simulink model "Simscape_Drone_Model"  (R2025b)
settings: Solver=FixedStepAuto  StartTime=0.0  StopTime=10  RelTol=1e-6  EnableMultiTasking=on
undefined symbols (not defined in the file): Aero_On, Config, P, SimParams, SimscapeParams, X, Y, Z
libraries: sm_lib x89, nesl_utility x71, fl_lib x18, sdl_lib x8, slpidlib x4, batteryecm_lib x1
(part 5 of 5)

== system Simscape_Drone_Model/Drone Mechanical/Motor Holder 4/Aero Dynamic Drag ==
  rho : Inport
  Gain : Gain  Gain=Aero_On
  MATLAB Function : MATLAB Function  TreatAsAtomicUnit=on
  Motor Holder Axis : Constant  Value=SimscapeParams.MotorHolderAxis
  Motor Holder Drag Matrix : Constant  Value=SimscapeParams.MotorHolderCd
  Motor Holder Length : Constant  Value=SimscapeParams.MotorHeight
  Motor Holder Radius : Constant  Value=SimscapeParams.MotorRadius
  Mux : Mux  Inputs=3
  PS-Simulink Converter : nesl_utility/PS-Simulink Converter  PhysicalDomain=network_engine_domain  SubClassName=ps_output  LeftPortType=input  RightPortType=output  PseudoPeriodic=off  Frequencies=[]  VectorFormat=inherit  Unit=inherit  AffineConversion=off
  PS-Simulink Converter1 : nesl_utility/PS-Simulink Converter  PhysicalDomain=network_engine_domain  SubClassName=ps_output  LeftPortType=input  RightPortType=output  PseudoPeriodic=off  Frequencies=[]  VectorFormat=inherit  Unit=inherit  AffineConversion=off
  PS-Simulink Converter2 : nesl_utility/PS-Simulink Converter  PhysicalDomain=network_engine_domain  SubClassName=ps_output  LeftPortType=input  RightPortType=output  PseudoPeriodic=off  Frequencies=[]  VectorFormat=inherit  Unit=inherit  AffineConversion=off
  Transform Sensor : sm_lib/Frames and Transforms/Transform Sensor  MeasurementFrame=NonRotatingFollower  RotationSequence=XYZ  SenseAngle=off  SenseAxis=off  SenseQ=off  SenseR=off  SenseRotationSequence=off  SenseOmegaX=off  SenseOmegaY=off  SenseOmegaZ=off  SenseOmega=off  SenseQDot=off  SenseRDot=off  SenseRotationSequenceDot=off  SenseAlphaX=off  SenseAlphaY=off  SenseAlphaZ=off  SenseAlpha=off  SenseQDDot=off  SenseRDDot=off  SenseX=off  SenseY=off  SenseZ=off  SenseXYZ=off  SenseRad=off  SenseAzim=off  SenseDist=off  SenseInc=off  SenseXDot=on  SenseYDot=on  SenseZDot=on  SenseXYZDot=off  SenseRadDot=off  SenseAzimDot=off  SenseDistDot=off  SenseIncDot=off  SenseXDDot=off  SenseYDDot=off  SenseZDDot=off  SenseXYZDDot=off  SenseRadDDot=off  SenseAzimDDot=off  SenseDistDDot=off  SenseIncDDot=off
  NED : PMIOPort  Side=Left
  F : PMIOPort  Port=2  Side=Left
  F_drag : Outport
  wires:
  PS-Simulink Converter/1 -> Mux/1
  PS-Simulink Converter2/1 -> Mux/3
  PS-Simulink Converter1/1 -> Mux/2
  rho/1 -> MATLAB Function/2(rho)
  Motor Holder Drag Matrix/1 -> MATLAB Function/3(Cd)
  Motor Holder Axis/1 -> MATLAB Function/6(axis)
  Motor Holder Radius/1 -> MATLAB Function/4(R)
  Motor Holder Length/1 -> MATLAB Function/5(L)
  Mux/1 -> MATLAB Function/1(v)
  MATLAB Function/1(F_drag) -> Gain/1
  Gain/1 -> F_drag/1
  connections:
  PS-Simulink Converter1/LConn1 -- Transform Sensor/RConn3
  PS-Simulink Converter2/LConn1 -- Transform Sensor/RConn4
  PS-Simulink Converter/LConn1 -- Transform Sensor/RConn2
  NED/RConn1 -- Transform Sensor/LConn1
  F/RConn1 -- Transform Sensor/RConn1

== system Simscape_Drone_Model/Drone Mechanical/Rotor arms/Subsystem ==
  note: Aero Dynamic Drag 2
  rho : Inport
  Arm Axis : Constant  Value=SimscapeParams.ArmAxis
  Arm Drag Matrix : Constant  Value=SimscapeParams.ArmCd
  Arm Length : Constant  Value=SimscapeParams.ArmLength
  Arm Radius : Constant  Value=SimscapeParams.ArmRadius
  Gain : Gain  Gain=Aero_On
  MATLAB Function : MATLAB Function  TreatAsAtomicUnit=on
  Mux : Mux  Inputs=3
  PS-Simulink Converter : nesl_utility/PS-Simulink Converter  PhysicalDomain=network_engine_domain  SubClassName=ps_output  LeftPortType=input  RightPortType=output  PseudoPeriodic=off  Frequencies=[]  VectorFormat=inherit  Unit=inherit  AffineConversion=off
  PS-Simulink Converter1 : nesl_utility/PS-Simulink Converter  PhysicalDomain=network_engine_domain  SubClassName=ps_output  LeftPortType=input  RightPortType=output  PseudoPeriodic=off  Frequencies=[]  VectorFormat=inherit  Unit=inherit  AffineConversion=off
  PS-Simulink Converter2 : nesl_utility/PS-Simulink Converter  PhysicalDomain=network_engine_domain  SubClassName=ps_output  LeftPortType=input  RightPortType=output  PseudoPeriodic=off  Frequencies=[]  VectorFormat=inherit  Unit=inherit  AffineConversion=off
  Transform Sensor : sm_lib/Frames and Transforms/Transform Sensor  MeasurementFrame=NonRotatingFollower  RotationSequence=XYZ  SenseAngle=off  SenseAxis=off  SenseQ=off  SenseR=off  SenseRotationSequence=off  SenseOmegaX=off  SenseOmegaY=off  SenseOmegaZ=off  SenseOmega=off  SenseQDot=off  SenseRDot=off  SenseRotationSequenceDot=off  SenseAlphaX=off  SenseAlphaY=off  SenseAlphaZ=off  SenseAlpha=off  SenseQDDot=off  SenseRDDot=off  SenseX=off  SenseY=off  SenseZ=off  SenseXYZ=off  SenseRad=off  SenseAzim=off  SenseDist=off  SenseInc=off  SenseXDot=on  SenseYDot=on  SenseZDot=on  SenseXYZDot=off  SenseRadDot=off  SenseAzimDot=off  SenseDistDot=off  SenseIncDot=off  SenseXDDot=off  SenseYDDot=off  SenseZDDot=off  SenseXYZDDot=off  SenseRadDDot=off  SenseAzimDDot=off  SenseDistDDot=off  SenseIncDDot=off
  NED : PMIOPort  Side=Left
  F : PMIOPort  Port=2  Side=Right
  F_drag : Outport
  wires:
  MATLAB Function/1(F_drag) -> Gain/1
  Mux/1 -> MATLAB Function/1(v)
  PS-Simulink Converter/1 -> Mux/1
  Arm Length/1 -> MATLAB Function/5(L)
  rho/1 -> MATLAB Function/2(rho)
  Arm Drag Matrix/1 -> MATLAB Function/3(Cd)
  PS-Simulink Converter2/1 -> Mux/3
  Arm Radius/1 -> MATLAB Function/4(R)
  PS-Simulink Converter1/1 -> Mux/2
  Arm Axis/1 -> MATLAB Function/6(axis)
  Gain/1 -> F_drag/1
  connections:
  PS-Simulink Converter/LConn1 -- Transform Sensor/RConn2
  PS-Simulink Converter1/LConn1 -- Transform Sensor/RConn3
  NED/RConn1 -- Transform Sensor/LConn1
  PS-Simulink Converter2/LConn1 -- Transform Sensor/RConn4
  F/RConn1 -- Transform Sensor/RConn1

== system Simscape_Drone_Model/Drone Mechanical/Rotor arms/Subsystem1 ==
  note: Aero Dynamic Drag 1
  rho : Inport
  Arm Axis : Constant  Value=SimscapeParams.ArmAxis
  Arm Drag Matrix : Constant  Value=SimscapeParams.ArmCd
  Arm Length : Constant  Value=SimscapeParams.ArmLength
  Arm Radius : Constant  Value=SimscapeParams.ArmRadius
  Gain : Gain  Gain=Aero_On
  MATLAB Function : MATLAB Function  TreatAsAtomicUnit=on
  Mux : Mux  Inputs=3
  PS-Simulink Converter : nesl_utility/PS-Simulink Converter  PhysicalDomain=network_engine_domain  SubClassName=ps_output  LeftPortType=input  RightPortType=output  PseudoPeriodic=off  Frequencies=[]  VectorFormat=inherit  Unit=inherit  AffineConversion=off
  PS-Simulink Converter1 : nesl_utility/PS-Simulink Converter  PhysicalDomain=network_engine_domain  SubClassName=ps_output  LeftPortType=input  RightPortType=output  PseudoPeriodic=off  Frequencies=[]  VectorFormat=inherit  Unit=inherit  AffineConversion=off
  PS-Simulink Converter2 : nesl_utility/PS-Simulink Converter  PhysicalDomain=network_engine_domain  SubClassName=ps_output  LeftPortType=input  RightPortType=output  PseudoPeriodic=off  Frequencies=[]  VectorFormat=inherit  Unit=inherit  AffineConversion=off
  Transform Sensor : sm_lib/Frames and Transforms/Transform Sensor  MeasurementFrame=NonRotatingFollower  RotationSequence=XYZ  SenseAngle=off  SenseAxis=off  SenseQ=off  SenseR=off  SenseRotationSequence=off  SenseOmegaX=off  SenseOmegaY=off  SenseOmegaZ=off  SenseOmega=off  SenseQDot=off  SenseRDot=off  SenseRotationSequenceDot=off  SenseAlphaX=off  SenseAlphaY=off  SenseAlphaZ=off  SenseAlpha=off  SenseQDDot=off  SenseRDDot=off  SenseX=off  SenseY=off  SenseZ=off  SenseXYZ=off  SenseRad=off  SenseAzim=off  SenseDist=off  SenseInc=off  SenseXDot=on  SenseYDot=on  SenseZDot=on  SenseXYZDot=off  SenseRadDot=off  SenseAzimDot=off  SenseDistDot=off  SenseIncDot=off  SenseXDDot=off  SenseYDDot=off  SenseZDDot=off  SenseXYZDDot=off  SenseRadDDot=off  SenseAzimDDot=off  SenseDistDDot=off  SenseIncDDot=off
  NED : PMIOPort  Side=Left
  F : PMIOPort  Port=2  Side=Right
  F_drag : Outport
  wires:
  MATLAB Function/1(F_drag) -> Gain/1
  Mux/1 -> MATLAB Function/1(v)
  PS-Simulink Converter/1 -> Mux/1
  Arm Length/1 -> MATLAB Function/5(L)
  rho/1 -> MATLAB Function/2(rho)
  Arm Drag Matrix/1 -> MATLAB Function/3(Cd)
  PS-Simulink Converter2/1 -> Mux/3
  Arm Radius/1 -> MATLAB Function/4(R)
  PS-Simulink Converter1/1 -> Mux/2
  Arm Axis/1 -> MATLAB Function/6(axis)
  Gain/1 -> F_drag/1
  connections:
  PS-Simulink Converter/LConn1 -- Transform Sensor/RConn2
  PS-Simulink Converter1/LConn1 -- Transform Sensor/RConn3
  NED/RConn1 -- Transform Sensor/LConn1
  PS-Simulink Converter2/LConn1 -- Transform Sensor/RConn4
  F/RConn1 -- Transform Sensor/RConn1

== system Simscape_Drone_Model/Drone Mechanical/Rotor arms/Subsystem2 ==
  note: Aero Dynamic Drag 4
  rho : Inport
  Arm Axis : Constant  Value=SimscapeParams.ArmAxis
  Arm Drag Matrix : Constant  Value=SimscapeParams.ArmCd
  Arm Length : Constant  Value=SimscapeParams.ArmLength
  Arm Radius : Constant  Value=SimscapeParams.ArmRadius
  Gain : Gain  Gain=Aero_On
  MATLAB Function : MATLAB Function  TreatAsAtomicUnit=on
  Mux : Mux  Inputs=3
  PS-Simulink Converter : nesl_utility/PS-Simulink Converter  PhysicalDomain=network_engine_domain  SubClassName=ps_output  LeftPortType=input  RightPortType=output  PseudoPeriodic=off  Frequencies=[]  VectorFormat=inherit  Unit=inherit  AffineConversion=off
  PS-Simulink Converter1 : nesl_utility/PS-Simulink Converter  PhysicalDomain=network_engine_domain  SubClassName=ps_output  LeftPortType=input  RightPortType=output  PseudoPeriodic=off  Frequencies=[]  VectorFormat=inherit  Unit=inherit  AffineConversion=off
  PS-Simulink Converter2 : nesl_utility/PS-Simulink Converter  PhysicalDomain=network_engine_domain  SubClassName=ps_output  LeftPortType=input  RightPortType=output  PseudoPeriodic=off  Frequencies=[]  VectorFormat=inherit  Unit=inherit  AffineConversion=off
  Transform Sensor : sm_lib/Frames and Transforms/Transform Sensor  MeasurementFrame=NonRotatingFollower  RotationSequence=XYZ  SenseAngle=off  SenseAxis=off  SenseQ=off  SenseR=off  SenseRotationSequence=off  SenseOmegaX=off  SenseOmegaY=off  SenseOmegaZ=off  SenseOmega=off  SenseQDot=off  SenseRDot=off  SenseRotationSequenceDot=off  SenseAlphaX=off  SenseAlphaY=off  SenseAlphaZ=off  SenseAlpha=off  SenseQDDot=off  SenseRDDot=off  SenseX=off  SenseY=off  SenseZ=off  SenseXYZ=off  SenseRad=off  SenseAzim=off  SenseDist=off  SenseInc=off  SenseXDot=on  SenseYDot=on  SenseZDot=on  SenseXYZDot=off  SenseRadDot=off  SenseAzimDot=off  SenseDistDot=off  SenseIncDot=off  SenseXDDot=off  SenseYDDot=off  SenseZDDot=off  SenseXYZDDot=off  SenseRadDDot=off  SenseAzimDDot=off  SenseDistDDot=off  SenseIncDDot=off
  NED : PMIOPort  Side=Left
  F : PMIOPort  Port=2  Side=Right
  F_drag : Outport
  wires:
  MATLAB Function/1(F_drag) -> Gain/1
  Mux/1 -> MATLAB Function/1(v)
  PS-Simulink Converter/1 -> Mux/1
  Arm Length/1 -> MATLAB Function/5(L)
  rho/1 -> MATLAB Function/2(rho)
  Arm Drag Matrix/1 -> MATLAB Function/3(Cd)
  PS-Simulink Converter2/1 -> Mux/3
  Arm Radius/1 -> MATLAB Function/4(R)
  PS-Simulink Converter1/1 -> Mux/2
  Arm Axis/1 -> MATLAB Function/6(axis)
  Gain/1 -> F_drag/1
  connections:
  PS-Simulink Converter/LConn1 -- Transform Sensor/RConn2
  PS-Simulink Converter1/LConn1 -- Transform Sensor/RConn3
  NED/RConn1 -- Transform Sensor/LConn1
  PS-Simulink Converter2/LConn1 -- Transform Sensor/RConn4
  F/RConn1 -- Transform Sensor/RConn1

== system Simscape_Drone_Model/Drone Mechanical/Rotor arms/Subsystem3 ==
  note: Aero Dynamic Drag 3
  rho : Inport
  Arm Axis : Constant  Value=SimscapeParams.ArmAxis
  Arm Drag Matrix : Constant  Value=SimscapeParams.ArmCd
  Arm Length : Constant  Value=SimscapeParams.ArmLength
  Arm Radius : Constant  Value=SimscapeParams.ArmRadius
  Gain : Gain  Gain=Aero_On
  MATLAB Function : MATLAB Function  TreatAsAtomicUnit=on
  Mux : Mux  Inputs=3
  PS-Simulink Converter : nesl_utility/PS-Simulink Converter  PhysicalDomain=network_engine_domain  SubClassName=ps_output  LeftPortType=input  RightPortType=output  PseudoPeriodic=off  Frequencies=[]  VectorFormat=inherit  Unit=inherit  AffineConversion=off
  PS-Simulink Converter1 : nesl_utility/PS-Simulink Converter  PhysicalDomain=network_engine_domain  SubClassName=ps_output  LeftPortType=input  RightPortType=output  PseudoPeriodic=off  Frequencies=[]  VectorFormat=inherit  Unit=inherit  AffineConversion=off
  PS-Simulink Converter2 : nesl_utility/PS-Simulink Converter  PhysicalDomain=network_engine_domain  SubClassName=ps_output  LeftPortType=input  RightPortType=output  PseudoPeriodic=off  Frequencies=[]  VectorFormat=inherit  Unit=inherit  AffineConversion=off
  Transform Sensor : sm_lib/Frames and Transforms/Transform Sensor  MeasurementFrame=NonRotatingFollower  RotationSequence=XYZ  SenseAngle=off  SenseAxis=off  SenseQ=off  SenseR=off  SenseRotationSequence=off  SenseOmegaX=off  SenseOmegaY=off  SenseOmegaZ=off  SenseOmega=off  SenseQDot=off  SenseRDot=off  SenseRotationSequenceDot=off  SenseAlphaX=off  SenseAlphaY=off  SenseAlphaZ=off  SenseAlpha=off  SenseQDDot=off  SenseRDDot=off  SenseX=off  SenseY=off  SenseZ=off  SenseXYZ=off  SenseRad=off  SenseAzim=off  SenseDist=off  SenseInc=off  SenseXDot=on  SenseYDot=on  SenseZDot=on  SenseXYZDot=off  SenseRadDot=off  SenseAzimDot=off  SenseDistDot=off  SenseIncDot=off  SenseXDDot=off  SenseYDDot=off  SenseZDDot=off  SenseXYZDDot=off  SenseRadDDot=off  SenseAzimDDot=off  SenseDistDDot=off  SenseIncDDot=off
  NED : PMIOPort  Side=Left
  F : PMIOPort  Port=2  Side=Right
  F_drag : Outport
  wires:
  MATLAB Function/1(F_drag) -> Gain/1
  Mux/1 -> MATLAB Function/1(v)
  PS-Simulink Converter/1 -> Mux/1
  Arm Length/1 -> MATLAB Function/5(L)
  rho/1 -> MATLAB Function/2(rho)
  Arm Drag Matrix/1 -> MATLAB Function/3(Cd)
  PS-Simulink Converter2/1 -> Mux/3
  Arm Radius/1 -> MATLAB Function/4(R)
  PS-Simulink Converter1/1 -> Mux/2
  Arm Axis/1 -> MATLAB Function/6(axis)
  Gain/1 -> F_drag/1
  connections:
  PS-Simulink Converter/LConn1 -- Transform Sensor/RConn2
  PS-Simulink Converter1/LConn1 -- Transform Sensor/RConn3
  NED/RConn1 -- Transform Sensor/LConn1
  PS-Simulink Converter2/LConn1 -- Transform Sensor/RConn4
  F/RConn1 -- Transform Sensor/RConn1

== system Simscape_Drone_Model/Drone Mechanical/Body/Top Payload/Top Payload ==
  rho : Inport
  Collsioin : Subsystem
  Cylindrical Solid : sm_lib/Body Elements/Cylindrical Solid  CylinderRadius=Config.TopPayload.Geometry.Radius  CylinderRadiusUnits=m  CylinderLength=Config.TopPayload.Geometry.Height  CylinderLengthUnits=m  ExportEntireGeometry=off  InertiaType=CalculateFromGeometry  BasedOnType=Mass  Density=1000  DensityUnits=kg/m^3  Mass=Config.TopPayload.Mass  MassUnits=kg  CenterOfMass=[0 0 0]  CenterOfMassUnits=m  MomentsOfInertia=[1 1 1]  MomentsOfInertiaUnits=kg*m^2  ProductsOfInertia=[0 0 0]  ProductsOfInertiaUnits=kg*m^2  GraphicType=FromGeometry  MarkerShape=Sphere  MarkerSize=10  GraphicVisPropType=SimpleVisualProperties  GraphicDiffuseColor=[1 0 1]  GraphicOpacity=1  GraphicSpecularColor=[0.5 0.5 0.5 1.0]  GraphicAmbientColor=[0.15 0.15 0.15 1.0]  GraphicEmissiveColor=[0.0 0.0 0.0 1.0]  GraphicShininess=75  DoExposeReferenceFrame=on  SerializedFrames=|
      | <Frames>
      | 
      |   <Frame>
      |     <Id>Frame1</Id>
      |     <Value>
      |       <Name>side</Name>
      |       <Origin>
      |         <Source>GeometricFeature</Source>
      |         <FeatureName>side surface</FeatureName>
      |       </Origin>
      |       <PrimaryAxis>
      |         <DefinedDirection>+Z</DefinedDirection>
      |         <Source>ReferenceFrame</Source>
      |         <SourceDirection>+Z</SourceDirection>
      |         <FeatureName></FeatureName>
      |       </PrimaryAxis>
      |       <SecondaryAxis>
      |         <DefinedDirection>+X</DefinedDirection>
      |         <Source>ReferenceFrame</Source>
      |         <SourceDirection>+X</SourceDirection>
      |         <FeatureName></FeatureName>
      |       </SecondaryAxis>
      |     </Value>
      |   </Frame>
      | 
      | </Frames>
  External Force and Torque1 : sm_lib/Forces and Torques/External Force and Torque  EnableForceX=off  EnableForceY=off  EnableForceZ=off  EnableForce=on  ForceResolutionFrame=AttachedFrame  EnableTorqueX=off  EnableTorqueY=off  EnableTorqueZ=off  EnableTorque=off  TorqueResolutionFrame=AttachedFrame
  Rigid Transform : sm_lib/Frames and Transforms/Rigid Transform  RotationMethod=None  FollAlignAxisA=+X  BaseAlignAxisA=+Y  FollAlignAxisB=+Y  BaseAlignAxisB=+Z  RotationStandardAxis=+Z  RotationAngle=0  RotationAngleUnits=deg  RotationArbitraryAxis=[0 0 1]  RotationSequenceAxes=FollowerAxes  RotationSequence=XYX  RotationSequenceAngles=[0 0 0]  RotationSequenceAnglesUnits=deg  RotationMatrix=[1 0 0;0 1 0;0 0 1]  Quaternion=[1 0 0 0]  TranslationMethod=Cartesian  TranslationCartesianOffset=[0 0 -(Config.Drone.Body_Height/2 + Config.TopPayload.Geometry.Height/2)]  TranslationCartesianOffsetUnits=m  TranslationStandardAxis=+Z  TranslationStandardOffset=0  TranslationStandardOffsetUnits=m  TranslationROffset=0  TranslationROffsetUnits=m  TranslationThetaOffset=0  TranslationThetaOffsetUnits=deg  TranslationZOffset=0  TranslationZOffsetUnits=m
  Simulink-PS Converter1 : nesl_utility/Simulink-PS Converter  PhysicalDomain=network_engine_domain  SubClassName=ps_input  LeftPortType=input  RightPortType=output  PseudoPeriodic=off  Frequencies=[]  NoiseDistribution=none  NoiseParameters=[]  Unit=N  AffineConversion=off  FilteringAndDerivatives=provide  SimscapeFilterOrder=1  InputFilterTimeConstant=0.001  UdotUserProvided=0
  Top payload drag : Subsystem
      settings: PortSchema="{\"entries\":[{\"content\":{\"sides\":[{\"content\":{\"connectorIds\":[\"LConn1\",\"In1\"]},\"type\":\"ConnectorPlacement.EquallySpacedRectSide\",\"uuid\":\"0fc06b31-134b-40cc-bbcb-bc6e67fd0f90\"},{\"content\":{\"connectorIds\":[\"RConn1\",\"Out1\"],\"side\":\"RIGHT\"},\"type\":\"ConnectorPlacement.EquallySpacedRectSide\",\"uuid\":\"8ba8f1df-0f30-4005-8c63-0e1ae2e2ce41\"},{\"content\":{\"side\":\"TOP\"},\"type\":\"ConnectorPlacement.EquallySpacedRectSide\",\"uuid\":\"8c63a784-8cbe-42b9-959e-29358ae8c9e6\"}]},\"type\":\"ConnectorPlacement.EquallySpacedConnector\",\"uuid\":\"fa01ef64-01b6-4a76-afbb-3e89d462b0f0\"}],\"packageUris\":[\"http://schema.mathworks.com/mf0/Connector/R2020b\"],\"version\":\"1.0\"}"
  Top Connection : PMIOPort  Side=Left
  NED : PMIOPort  Port=2  Side=Left
  Body Collision : PMIOPort  Port=3  Side=Left
  wires:
  Top payload drag/1(F_drag) -> Simulink-PS Converter1/1
  rho/1 -> Top payload drag/1(rho)
  connections:
  External Force and Torque1/LConn1 -- Simulink-PS Converter1/RConn1
  Cylindrical Solid/RConn1 -- Rigid Transform/RConn1 -- External Force and Torque1/RConn1 -- Top payload drag/RConn1
  Rigid Transform/LConn1 -- Top Connection/RConn1
  Top payload drag/LConn1 -- NED/RConn1
  Collsioin/LConn1 -- Cylindrical Solid/LConn1
  Body Collision/RConn1 -- Collsioin/RConn1

== system Simscape_Drone_Model/Drone Mechanical/Body/Top Payload/Top Payload/Collsioin ==
  PS-Simulink Converter : nesl_utility/PS-Simulink Converter  PhysicalDomain=network_engine_domain  SubClassName=ps_output  LeftPortType=input  RightPortType=output  PseudoPeriodic=off  Frequencies=[]  VectorFormat=inherit  Unit=inherit  AffineConversion=off
  PS-Simulink Converter1 : nesl_utility/PS-Simulink Converter  PhysicalDomain=network_engine_domain  SubClassName=ps_output  LeftPortType=input  RightPortType=output  PseudoPeriodic=off  Frequencies=[]  VectorFormat=inherit  Unit=inherit  AffineConversion=off
  PS-Simulink Converter2 : nesl_utility/PS-Simulink Converter  PhysicalDomain=network_engine_domain  SubClassName=ps_output  LeftPortType=input  RightPortType=output  PseudoPeriodic=off  Frequencies=[]  VectorFormat=inherit  Unit=inherit  AffineConversion=off
  Point Cloud : sm_lib/Curves and Surfaces/Point Cloud  CoordinatesMatrix=SimscapeParams.TopPayloadSurfacePoints  CoordinatesMatrixUnits=m  GraphicType=MarkerCloud  GraphicSphereRadius=1e-2  GraphicSphereRadiusUnits=m  GraphicVisPropType=SimpleVisualProperties  GraphicDiffuseColor=[0.5 0.5 0.5]  GraphicOpacity=1  GraphicSpecularColor=[0.5 0.5 0.5 1.0]  GraphicAmbientColor=[0.15 0.15 0.15 1.0]  GraphicEmissiveColor=[0.0 0.0 0.0 1.0]  GraphicShininess=75
  Scope : Scope  Commented=on  NumInputPorts=3
      settings: ActiveDisplayYMinimum=-0.12499999999999997  ActiveDisplayYMaximum=1.125  DataLoggingVariableName=ScopeData3
  Spatial Contact Force1 : sm_lib/Forces and Torques/Spatial Contact Force  SenseSeparationDistance=off  NormalForceType=SmoothSpringDamper  NormalStiffness=2.5e4  NormalStiffnessUnits=N/m  NormalDamping=50  NormalDampingUnits=N/(m/s)  NormalTransitionRegionWidth=1e-3  NormalTransitionRegionWidthUnits=m  FrictionType=None  CoefficientOfStaticFriction=0.8  CoefficientOfDynamicFriction=0.5  FrictionalCriticalVelocity=1e-2  FrictionalCriticalVelocityUnits=m/s  SenseContactSignal=on  SensePenetrationDepth=off  SenseNormalVelocity=off  SenseTangentialVelocity=on  SensingForceTorqueDirection=BaseOnFollower  SensingForceTorqueResolutionFrame=BaseFrame  SenseNormalForce=off  SenseNormalForceMagnitude=off  SenseNormalTorque=off  SenseFrictionalForce=on  SenseFrictionalForceMagnitude=off  SenseFrictionalTorque=off  SenseTotalForce=off  SenseTotalTorque=off  SenseContactBaseRotation=off  SenseContactBaseTranslation=off  SenseContactFollowerRotation=off  SenseContactFollowerTranslation=off  ZeroCrossDetectContactStartAndEnd=off
  Side : PMIOPort  Side=Left
  Body Collision : PMIOPort  Port=2  Side=Right
  wires:
  PS-Simulink Converter2/1 -> Scope/3  "Tangential Velocity"
  PS-Simulink Converter1/1 -> Scope/2  "Frictional Force"
  PS-Simulink Converter/1 -> Scope/1  "Contact"
  connections:
  PS-Simulink Converter2/LConn1 -- Spatial Contact Force1/RConn4
  PS-Simulink Converter1/LConn1 -- Spatial Contact Force1/RConn3
  PS-Simulink Converter/LConn1 -- Spatial Contact Force1/RConn2
  Side/RConn1 -- Point Cloud/LConn1
  Spatial Contact Force1/LConn1 -- Point Cloud/RConn1
  Spatial Contact Force1/RConn1 -- Body Collision/RConn1

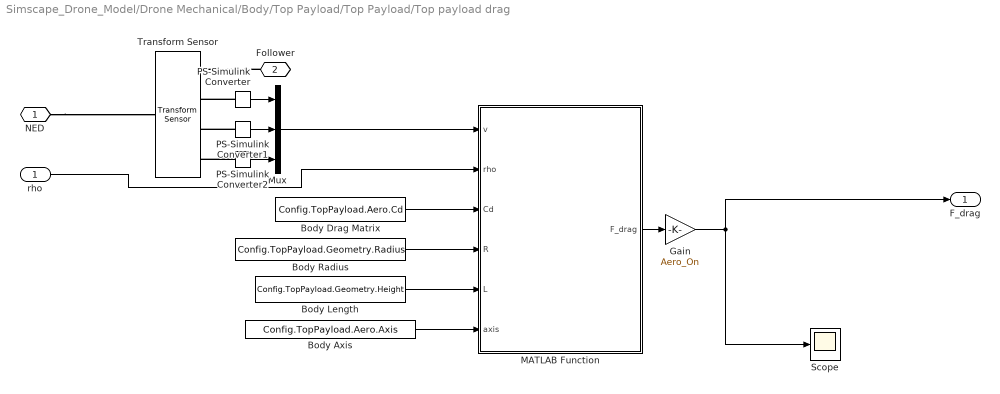
== system Simscape_Drone_Model/Drone Mechanical/Body/Top Payload/Top Payload/Top payload drag ==
  rho : Inport
  Body Axis : Constant  Value=Config.TopPayload.Aero.Axis
  Body Drag Matrix : Constant  Value=Config.TopPayload.Aero.Cd
  Body Length : Constant  Value=Config.TopPayload.Geometry.Height
  Body Radius : Constant  Value=Config.TopPayload.Geometry.Radius
  Gain : Gain  Gain=Aero_On
  MATLAB Function : MATLAB Function  TreatAsAtomicUnit=on
  Mux : Mux  Inputs=3
  PS-Simulink Converter : nesl_utility/PS-Simulink Converter  PhysicalDomain=network_engine_domain  SubClassName=ps_output  LeftPortType=input  RightPortType=output  PseudoPeriodic=off  Frequencies=[]  VectorFormat=inherit  Unit=inherit  AffineConversion=off
  PS-Simulink Converter1 : nesl_utility/PS-Simulink Converter  PhysicalDomain=network_engine_domain  SubClassName=ps_output  LeftPortType=input  RightPortType=output  PseudoPeriodic=off  Frequencies=[]  VectorFormat=inherit  Unit=inherit  AffineConversion=off
  PS-Simulink Converter2 : nesl_utility/PS-Simulink Converter  PhysicalDomain=network_engine_domain  SubClassName=ps_output  LeftPortType=input  RightPortType=output  PseudoPeriodic=off  Frequencies=[]  VectorFormat=inherit  Unit=inherit  AffineConversion=off
  Scope : Scope
      settings: ActiveDisplayYMinimum=-1  ActiveDisplayYMaximum=1  DataLoggingVariableName=ScopeData4
  Transform Sensor : sm_lib/Frames and Transforms/Transform Sensor  MeasurementFrame=NonRotatingFollower  RotationSequence=XYZ  SenseAngle=off  SenseAxis=off  SenseQ=off  SenseR=off  SenseRotationSequence=off  SenseOmegaX=off  SenseOmegaY=off  SenseOmegaZ=off  SenseOmega=off  SenseQDot=off  SenseRDot=off  SenseRotationSequenceDot=off  SenseAlphaX=off  SenseAlphaY=off  SenseAlphaZ=off  SenseAlpha=off  SenseQDDot=off  SenseRDDot=off  SenseX=off  SenseY=off  SenseZ=off  SenseXYZ=off  SenseRad=off  SenseAzim=off  SenseDist=off  SenseInc=off  SenseXDot=on  SenseYDot=on  SenseZDot=on  SenseXYZDot=off  SenseRadDot=off  SenseAzimDot=off  SenseDistDot=off  SenseIncDot=off  SenseXDDot=off  SenseYDDot=off  SenseZDDot=off  SenseXYZDDot=off  SenseRadDDot=off  SenseAzimDDot=off  SenseDistDDot=off  SenseIncDDot=off
  NED : PMIOPort  Side=Left
  Follower : PMIOPort  Port=2  Side=Right
  F_drag : Outport
  wires:
  Body Axis/1 -> MATLAB Function/6(axis)
  Body Drag Matrix/1 -> MATLAB Function/3(Cd)
  PS-Simulink Converter/1 -> Mux/1
  PS-Simulink Converter1/1 -> Mux/2
  Body Radius/1 -> MATLAB Function/4(R)
  Body Length/1 -> MATLAB Function/5(L)
  MATLAB Function/1(F_drag) -> Gain/1
  rho/1 -> MATLAB Function/2(rho)
  PS-Simulink Converter2/1 -> Mux/3
  Mux/1 -> MATLAB Function/1(v)
  Gain/1 -> F_drag/1, Scope/1
  connections:
  PS-Simulink Converter2/LConn1 -- Transform Sensor/RConn4
  PS-Simulink Converter1/LConn1 -- Transform Sensor/RConn3
  NED/RConn1 -- Transform Sensor/LConn1
  Follower/RConn1 -- Transform Sensor/RConn1
  PS-Simulink Converter/LConn1 -- Transform Sensor/RConn2

== matlab function Simscape_Drone_Model/Drone Mechanical/Rotor arms/Subsystem3/MATLAB Function ==
  data: v input; F_drag output; rho input; Cd input; R input; L input; axis input
function F_drag = cylinder_drag(v, rho, Cd, R, L, axis)
%#codegen
%
% axis = unit vector representing cylinder axis
% in the local measurement frame.

speed = sqrt(v(1)^2 + v(2)^2 + v(3)^2);

if speed < 1e-6
    F_drag = zeros(3,1);
    return;
end

v_hat = v / speed;

cos_theta = abs( ...
    v_hat(1)*axis(1) + ...
    v_hat(2)*axis(2) + ...
    v_hat(3)*axis(3));

cos_theta = min(max(cos_theta,0),1);

sin_theta = sqrt(1 - cos_theta^2);

A_proj = ...
    2*R*L*sin_theta + ...
    pi*R^2*cos_theta;

F_drag = -0.5*rho*Cd*A_proj*speed*v;

end

== matlab function Simscape_Drone_Model/Drone Mechanical/Rotor arms/Subsystem2/MATLAB Function ==
  data: v input; F_drag output; rho input; Cd input; R input; L input; axis input
function F_drag = cylinder_drag(v, rho, Cd, R, L, axis)
%#codegen
%
% axis = unit vector representing cylinder axis
% in the local measurement frame.

speed = sqrt(v(1)^2 + v(2)^2 + v(3)^2);

if speed < 1e-6
    F_drag = zeros(3,1);
    return;
end

v_hat = v / speed;

cos_theta = abs( ...
    v_hat(1)*axis(1) + ...
    v_hat(2)*axis(2) + ...
    v_hat(3)*axis(3));

cos_theta = min(max(cos_theta,0),1);

sin_theta = sqrt(1 - cos_theta^2);

A_proj = ...
    2*R*L*sin_theta + ...
    pi*R^2*cos_theta;

F_drag = -0.5*rho*Cd*A_proj*speed*v;

end

== matlab function Simscape_Drone_Model/ENU to NED/MATLAB Function ==
  data: S_base input; S_ned output; Sdot_base input; Sddot_base input; Omega_base input; Eta_in input; R_raw input; Sdot_ned output; Sddot_ned output; Omega_frd output; Omega_nav_ned output; Eta_ned output; R_ned output; R_ned_to_frd output
function [S_ned, Sdot_ned, Sddot_ned, ...
          Omega_frd, Omega_nav_ned, ...
          Eta_ned, R_ned, R_ned_to_frd] = ...
    drone2ideal_ned(S_base, Sdot_base, Sddot_base, ...
                    Omega_base, Eta_in, R_raw)

%#codegen
%
% Simscape World:
%   ENU
%       +X = East
%       +Y = North
%       +Z = Up
%
% PX4 navigation:
%   NED
%       +X = North
%       +Y = East
%       +Z = Down
%
% IMPORTANT:
%
% Transform Sensor:
%   B = NED frame
%   F = drone body
%
% R_raw already maps:
%
%       drone body -> NED
%
% Therefore NO additional body-frame conversion is required.


%% ENU World -> NED

T_enu_to_ned = [0  1  0;
                1  0  0;
                0  0 -1];


%% Local position origin

persistent S0

if isempty(S0)
    S0 = S_base;
end


%% Translation
%
% Transform Sensor Measurement Frame = World.
%
% These quantities are therefore expressed in the Simscape
% World frame (ENU) and must be converted to NED.

S_ned = T_enu_to_ned * (S_base - S0);

Sdot_ned = T_enu_to_ned * Sdot_base;

Sddot_ned = T_enu_to_ned * Sddot_base;


%% Attitude
%
% R_raw already maps:
%
%       body -> NED
%
% Do NOT apply ENU->NED here.
% Do NOT apply FLU->FRD here.

R_ned = R_raw;


%% NED -> body

R_ned_to_frd = R_ned.';


%% Angular velocity
%
% Measurement Frame = World, so Omega_base is expressed
% in ENU coordinates.

Omega_nav_ned = T_enu_to_ned * Omega_base;


%% NED-resolved angular velocity -> body coordinates

Omega_frd = R_ned_to_frd * Omega_nav_ned;


%% Euler angles
%
% R_ned = body -> NED
%
% Standard ZYX decomposition

theta_ned = asin_sat(-R_ned(3,1));

phi_ned = atan2( ...
    R_ned(3,2), ...
    R_ned(3,3));

psi_ned = atan2( ...
    R_ned(2,1), ...
    R_ned(1,1));


%% Order for Rotation Angles to Quaternions block
%
% Block is configured ZYX:
%
%   [yaw;
%    pitch;
%    roll]

Eta_ned = [psi_ned;
           theta_ned;
           phi_ned];


%% Eta_in intentionally unused

end


function y = asin_sat(x)
%#codegen

x = min(max(x,-1),1);
y = asin(x);

end

== matlab function Simscape_Drone_Model/Drone Mechanical/Motor Holder 2/Aero Dynamic Drag/MATLAB Function ==
  data: v input; F_drag output; rho input; Cd input; R input; L input; axis input
function F_drag = cylinder_drag(v, rho, Cd, R, L, axis)
%#codegen
%
% axis = unit vector representing cylinder axis
% in the local measurement frame.

speed = sqrt(v(1)^2 + v(2)^2 + v(3)^2);

if speed < 1e-6
    F_drag = zeros(3,1);
    return;
end

v_hat = v / speed;

cos_theta = abs( ...
    v_hat(1)*axis(1) + ...
    v_hat(2)*axis(2) + ...
    v_hat(3)*axis(3));

cos_theta = min(max(cos_theta,0),1);

sin_theta = sqrt(1 - cos_theta^2);

A_proj = ...
    2*R*L*sin_theta + ...
    pi*R^2*cos_theta;

F_drag = -0.5*rho*Cd*A_proj*speed*v;

end

== matlab function Simscape_Drone_Model/MATLAB Function1 ==
  data: h input; rho output
function rho  = isa_atmosphere(h)
%#codegen
% ISA atmosphere model for the troposphere.
%
% Input:
%   h   Altitude above mean sea level [m]
%
% Outputs:
%   T   Temperature [K]
%   a   Speed of sound [m/s]
%   P   Atmospheric pressure [Pa]
%   rho Air density [kg/m^3]

% ISA sea-level constants
T0    = 288.15;       % [K]
P0    = 101325.0;     % [Pa]
g0    = 9.80665;      % [m/s^2]
R_air = 287.05287;    % [J/(kg*K)]
L     = 0.0065;       % [K/m], temperature lapse rate

% Keep the model inside the troposphere validity range
h = min(max(h, -500.0), 11000.0);

% ISA temperature
T = T0 - L*h;

% ISA pressure
P = P0*(T/T0)^(g0/(R_air*L));

% Ideal-gas density
rho = P/(R_air*T);

end

== matlab function Simscape_Drone_Model/Drone Mechanical/Rotor arms/Subsystem/MATLAB Function ==
  data: v input; F_drag output; rho input; Cd input; R input; L input; axis input
function F_drag = cylinder_drag(v, rho, Cd, R, L, axis)
%#codegen
%
% axis = unit vector representing cylinder axis
% in the local measurement frame.

speed = sqrt(v(1)^2 + v(2)^2 + v(3)^2);

if speed < 1e-6
    F_drag = zeros(3,1);
    return;
end

v_hat = v / speed;

cos_theta = abs( ...
    v_hat(1)*axis(1) + ...
    v_hat(2)*axis(2) + ...
    v_hat(3)*axis(3));

cos_theta = min(max(cos_theta,0),1);

sin_theta = sqrt(1 - cos_theta^2);

A_proj = ...
    2*R*L*sin_theta + ...
    pi*R^2*cos_theta;

F_drag = -0.5*rho*Cd*A_proj*speed*v;

end

== matlab function Simscape_Drone_Model/Drone Mechanical/Body/Aero Dynamic Drag/MATLAB Function ==
  data: v input; F_drag output; rho input; Cd input; R input; L input; axis input
function F_drag = cylinder_drag(v, rho, Cd, R, L, axis)
%#codegen
%
% axis = unit vector representing cylinder axis
% in the local measurement frame.

speed = sqrt(v(1)^2 + v(2)^2 + v(3)^2);

if speed < 1e-6
    F_drag = zeros(3,1);
    return;
end

v_hat = v / speed;

cos_theta = abs( ...
    v_hat(1)*axis(1) + ...
    v_hat(2)*axis(2) + ...
    v_hat(3)*axis(3));

cos_theta = min(max(cos_theta,0),1);

sin_theta = sqrt(1 - cos_theta^2);

A_proj = ...
    2*R*L*sin_theta + ...
    pi*R^2*cos_theta;

F_drag = -0.5*rho*Cd*A_proj*speed*v;

end

== matlab function Simscape_Drone_Model/Drone Mechanical/Rotor arms/Subsystem1/MATLAB Function ==
  data: v input; F_drag output; rho input; Cd input; R input; L input; axis input
function F_drag = cylinder_drag(v, rho, Cd, R, L, axis)
%#codegen
%
% axis = unit vector representing cylinder axis
% in the local measurement frame.

speed = sqrt(v(1)^2 + v(2)^2 + v(3)^2);

if speed < 1e-6
    F_drag = zeros(3,1);
    return;
end

v_hat = v / speed;

cos_theta = abs( ...
    v_hat(1)*axis(1) + ...
    v_hat(2)*axis(2) + ...
    v_hat(3)*axis(3));

cos_theta = min(max(cos_theta,0),1);

sin_theta = sqrt(1 - cos_theta^2);

A_proj = ...
    2*R*L*sin_theta + ...
    pi*R^2*cos_theta;

F_drag = -0.5*rho*Cd*A_proj*speed*v;

end

== matlab function Simscape_Drone_Model/Drone Mechanical/Motor Holder 4/Aero Dynamic Drag/MATLAB Function ==
  data: v input; F_drag output; rho input; Cd input; R input; L input; axis input
function F_drag = cylinder_drag(v, rho, Cd, R, L, axis)
%#codegen
%
% axis = unit vector representing cylinder axis
% in the local measurement frame.

speed = sqrt(v(1)^2 + v(2)^2 + v(3)^2);

if speed < 1e-6
    F_drag = zeros(3,1);
    return;
end

v_hat = v / speed;

cos_theta = abs( ...
    v_hat(1)*axis(1) + ...
    v_hat(2)*axis(2) + ...
    v_hat(3)*axis(3));

cos_theta = min(max(cos_theta,0),1);

sin_theta = sqrt(1 - cos_theta^2);

A_proj = ...
    2*R*L*sin_theta + ...
    pi*R^2*cos_theta;

F_drag = -0.5*rho*Cd*A_proj*speed*v;

end

== matlab function Simscape_Drone_Model/Drone Mechanical/Motor Holder 1/Subsystem/MATLAB Function ==
  data: v input; F_drag output; rho input; Cd input; R input; L input; axis input
function F_drag = cylinder_drag(v, rho, Cd, R, L, axis)
%#codegen
%
% axis = unit vector representing cylinder axis
% in the local measurement frame.

speed = sqrt(v(1)^2 + v(2)^2 + v(3)^2);

if speed < 1e-6
    F_drag = zeros(3,1);
    return;
end

v_hat = v / speed;

cos_theta = abs( ...
    v_hat(1)*axis(1) + ...
    v_hat(2)*axis(2) + ...
    v_hat(3)*axis(3));

cos_theta = min(max(cos_theta,0),1);

sin_theta = sqrt(1 - cos_theta^2);

A_proj = ...
    2*R*L*sin_theta + ...
    pi*R^2*cos_theta;

F_drag = -0.5*rho*Cd*A_proj*speed*v;

end

== matlab function Simscape_Drone_Model/Drone Mechanical/Motor Holder 3/Aero Dynamic Drag/MATLAB Function ==
  data: v input; F_drag output; rho input; Cd input; R input; L input; axis input
function F_drag = cylinder_drag(v, rho, Cd, R, L, axis)
%#codegen
%
% axis = unit vector representing cylinder axis
% in the local measurement frame.

speed = sqrt(v(1)^2 + v(2)^2 + v(3)^2);

if speed < 1e-6
    F_drag = zeros(3,1);
    return;
end

v_hat = v / speed;

cos_theta = abs( ...
    v_hat(1)*axis(1) + ...
    v_hat(2)*axis(2) + ...
    v_hat(3)*axis(3));

cos_theta = min(max(cos_theta,0),1);

sin_theta = sqrt(1 - cos_theta^2);

A_proj = ...
    2*R*L*sin_theta + ...
    pi*R^2*cos_theta;

F_drag = -0.5*rho*Cd*A_proj*speed*v;

end

== matlab function Simscape_Drone_Model/Drone Mechanical/Body/Top Payload/Top Payload/Top payload drag/MATLAB Function ==
  data: v input; F_drag output; rho input; Cd input; R input; L input; axis input
function F_drag = cylinder_drag(v, rho, Cd, R, L, axis)
%#codegen
%
% axis = unit vector representing cylinder axis
% in the local measurement frame.

speed = sqrt(v(1)^2 + v(2)^2 + v(3)^2);

if speed < 1e-6
    F_drag = zeros(3,1);
    return;
end

v_hat = v / speed;

cos_theta = abs( ...
    v_hat(1)*axis(1) + ...
    v_hat(2)*axis(2) + ...
    v_hat(3)*axis(3));

cos_theta = min(max(cos_theta,0),1);

sin_theta = sqrt(1 - cos_theta^2);

A_proj = ...
    2*R*L*sin_theta + ...
    pi*R^2*cos_theta;

F_drag = -0.5*rho*Cd*A_proj*speed*v;

end
